simulink library "casper_library_pfbs"  (Simulink 7.2)
settings: Solver=ode45  SolverMode=SingleTasking  StartTime=0.0  StopTime=10.0  RelTol=1e-3
undefined symbols (not defined in the file or in its folder): pfb_coeff_gen_calc
libraries: xbsIndex_r4 x138, casper_library_pfbs x18, casper_library_delays x9, casper_library_misc x7, casper_library_flow_control x2
(part 2 of 3)

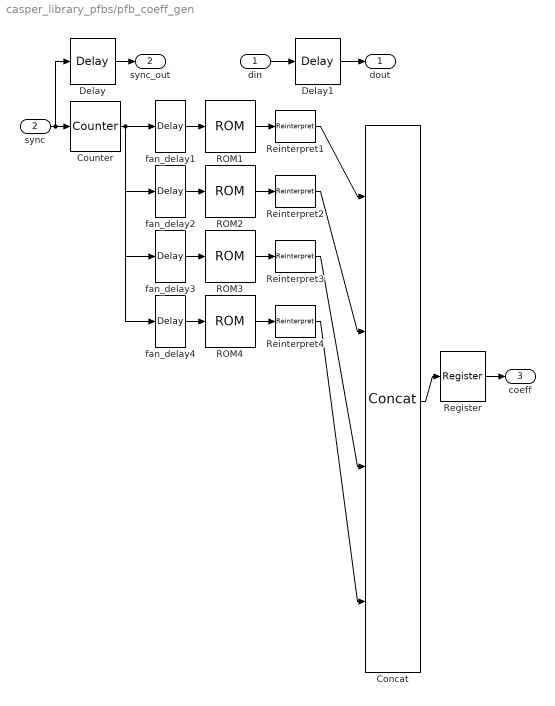
== system casper_library_pfbs/pfb_coeff_gen ==
  din : Inport
  sync : Inport  Port=2
  Concat : xbsIndex_r4/Concat  num_inputs=4  dbl_ovrd=off  block_type=concat
      settings: block_version=9.1.01
  Counter : xbsIndex_r4/Counter  cnt_type=Free Running  cnt_to=Inf  operation=Up  start_count=0  cnt_by_val=1  arith_type=Unsigned  n_bits=2  bin_pt=0  load_pin=off  rst=on  en=off  explicit_period=on  period=1  dbl_ovrd=off  use_behavioral_HDL=off  implementation=Fabric  use_rpm=on  block_type=counter
      settings: xl_area=[0, 0, 0, 0, 0, 0, 0]  block_version=9.1.01
  Delay : xbsIndex_r4/Delay  rst=off  infoeditControl=Selection of Reset will increase slice count due to use of real FFs and instead of SRLs  en=off  latency=bram_latency+1+fan_latency  dbl_ovrd=off  reg_retiming=off  block_type=delay
      settings: xl_area=[0, 0, 0, 0, 0, 0, 0]  block_version=9.1.01
  Delay1 : xbsIndex_r4/Delay  rst=off  infoeditControl=Selection of Reset will increase slice count due to use of real FFs and instead of SRLs  en=off  latency=bram_latency+1+fan_latency  dbl_ovrd=off  reg_retiming=off  block_type=delay
      settings: xl_area=[0, 0, 0, 0, 0, 0, 0]  block_version=9.1.01
  ROM1 : xbsIndex_r4/ROM  depth=4  initVector=pfb_coeff_gen_calc(2, 4,'hamming',0, 0,1,1,false)  distributed_mem=Block RAM  rst=off  init_reg=0  en=off  latency=bram_latency  gui_display_data_type=Fixed-point  arith_type="Signed  (2's comp)"  n_bits=8  bin_pt=7  preci_type=Single  exp_width=8  frac_width=24  dbl_ovrd=off  optimize=Area  use_rpm=on  block_type=sprom
      settings: xl_area=[0, 0, 0, 0, 0, 0, 0]
  ROM2 : xbsIndex_r4/ROM  depth=4  initVector=pfb_coeff_gen_calc(2, 4,'hamming',0, 0,1,2,false)  distributed_mem=Block RAM  rst=off  init_reg=0  en=off  latency=bram_latency  gui_display_data_type=Fixed-point  arith_type="Signed  (2's comp)"  n_bits=8  bin_pt=7  preci_type=Single  exp_width=8  frac_width=24  dbl_ovrd=off  optimize=Area  use_rpm=on  block_type=sprom
      settings: xl_area=[0, 0, 0, 0, 0, 0, 0]
  ROM3 : xbsIndex_r4/ROM  depth=4  initVector=pfb_coeff_gen_calc(2, 4,'hamming',0, 0,1,3,false)  distributed_mem=Block RAM  rst=off  init_reg=0  en=off  latency=bram_latency  gui_display_data_type=Fixed-point  arith_type="Signed  (2's comp)"  n_bits=8  bin_pt=7  preci_type=Single  exp_width=8  frac_width=24  dbl_ovrd=off  optimize=Area  use_rpm=on  block_type=sprom
      settings: xl_area=[0, 0, 0, 0, 0, 0, 0]
  ROM4 : xbsIndex_r4/ROM  depth=4  initVector=pfb_coeff_gen_calc(2, 4,'hamming',0, 0,1,4,false)  distributed_mem=Block RAM  rst=off  init_reg=0  en=off  latency=bram_latency  gui_display_data_type=Fixed-point  arith_type="Signed  (2's comp)"  n_bits=8  bin_pt=7  preci_type=Single  exp_width=8  frac_width=24  dbl_ovrd=off  optimize=Area  use_rpm=on  block_type=sprom
      settings: xl_area=[0, 0, 0, 0, 0, 0, 0]
  Register : xbsIndex_r4/Register  init=0  rst=off  en=off  dbl_ovrd=off  block_type=register
      settings: xl_area=[0, 0, 0, 0, 0, 0, 0]  block_version=9.1.01
  Reinterpret{1..4} (4 alike) : xbsIndex_r4/Reinterpret  force_arith_type=on  arith_type=Unsigned  force_bin_pt=on  bin_pt=0  block_type=reinterpret
      settings: infoedit="Changes signal type without altering the binary representation.   You can changed the signal between signed and unsigned, and relocate the binary point.<P><P>Hardware notes: In hardware this block costs nothing.<P><P>Example:  Suppose the input is 6 bits wide, signed, with 2 fractional bits, and the output is forced to unsigned with 0 fractional bits.  Then an input of -2.0 (1110.00 in binary 2's complement) becomes an output of 56 (111000 in binary)."  block_version=9.1.01
  fan_delay{1..4} (4 alike) : xbsIndex_r4/Delay  rst=off  infoeditControl=Selection of Reset will increase slice count due to use of real FFs and instead of SRLs  en=off  latency=fan_latency  dbl_ovrd=off  reg_retiming=off  block_type=delay
      settings: block_version=11.4
  dout : Outport
  sync_out : Outport  Port=2
  coeff : Outport  Port=3
  wires:
  din/1 -> Delay1/1
  Delay1/1 -> dout/1
  sync/1 -> Counter/1, Delay/1
  Delay/1 -> sync_out/1
  Concat/1 -> Register/1
  Register/1 -> coeff/1
  Counter/1 -> fan_delay1/1, fan_delay2/1, fan_delay3/1, fan_delay4/1
  fan_delay1/1 -> ROM1/1
  ROM1/1 -> Reinterpret1/1
  Reinterpret1/1 -> Concat/1
  fan_delay2/1 -> ROM2/1
  ROM2/1 -> Reinterpret2/1
  Reinterpret2/1 -> Concat/2
  fan_delay3/1 -> ROM3/1
  ROM3/1 -> Reinterpret3/1
  Reinterpret3/1 -> Concat/3
  fan_delay4/1 -> ROM4/1
  ROM4/1 -> Reinterpret4/1
  Reinterpret4/1 -> Concat/4

== system casper_library_pfbs/pfb_fir ==
  sync : Inport
  pol1_in1 : Inport  Port=2
  pol1_in2 : Inport  Port=3
  pol1_in1_coeffs : casper_library_pfbs/pfb_coeff_gen  PFBSize=5  CoeffBitWidth=18  TotalTaps=2  CoeffDistMem=off  WindowType=hamming  bram_latency=2  n_inputs=1  nput=0  fwidth=1  debug_mode=off  fan_latency=1
      settings: AttributesFormatString=|
      | PFBSize=5, n_inputs=1,
      | taps=2, input=0
  pol1_in1_first_tap : casper_library_pfbs/first_tap  PFBSize=5  CoeffBitWidth=18  TotalTaps=2  BitWidthIn=8  WindowType=hamming  mult_latency=2  bram_latency=2  n_inputs=1  fwidth=1  use_hdl=on  use_embedded=off
      settings: AttributesFormatString=taps=2
  pol1_in1_last_tap : casper_library_pfbs/last_tap  TotalTaps=2  BitWidthIn=8  BitWidthOut=18  CoeffBitWidth=18  add_latency=1  mult_latency=2  quantization="Round  (unbiased: Even Values)"  use_hdl=on  use_embedded=off
      link override pfb_add_tree/adder_tree1/addr1: latency=1  precision=User Defined  arith_type="Signed  (2's comp)"  n_bits=26  bin_pt=24  quantization=Truncate  overflow=Wrap  use_behavioral_HDL=off  hw_selection=Fabric  pipelined=on  use_rpm=on
      link override pfb_add_tree/adder_tree1/addr3: latency=1  precision=User Defined  arith_type="Signed  (2's comp)"  n_bits=26  bin_pt=24  quantization=Truncate  overflow=Wrap  use_behavioral_HDL=off  hw_selection=Fabric  pipelined=on  use_rpm=on
      link override pfb_add_tree/adder_tree2/addr1: latency=1  precision=User Defined  arith_type="Signed  (2's comp)"  n_bits=26  bin_pt=24  quantization=Truncate  overflow=Wrap  use_behavioral_HDL=off  hw_selection=Fabric  pipelined=on  use_rpm=on
      link override pfb_add_tree/adder_tree2/addr3: latency=1  precision=User Defined  arith_type="Signed  (2's comp)"  n_bits=26  bin_pt=24  quantization=Truncate  overflow=Wrap  use_behavioral_HDL=off  hw_selection=Fabric  pipelined=on  use_rpm=on
      link override pfb_add_tree/convert1: arith_type="Signed  (2's comp)"  n_bits=18  bin_pt=17  quantization="Round  (unbiased: Even Values)"  overflow=Wrap  latency=1  pipeline=on
      link override pfb_add_tree/convert2: arith_type="Signed  (2's comp)"  n_bits=18  bin_pt=17  quantization="Round  (unbiased: Even Values)"  overflow=Wrap  latency=1
      link override pfb_add_tree/scale1: scale_factor=-1
      link override pfb_add_tree/scale2: scale_factor=-1
      settings: AttributesFormatString=taps=2
  pol1_in2_coeffs : casper_library_pfbs/pfb_coeff_gen  PFBSize=5  CoeffBitWidth=18  TotalTaps=2  CoeffDistMem=off  WindowType=hamming  bram_latency=2  n_inputs=1  nput=1  fwidth=1  debug_mode=off  fan_latency=1
      settings: AttributesFormatString=|
      | PFBSize=5, n_inputs=1,
      | taps=2, input=1
  pol1_in2_first_tap : casper_library_pfbs/first_tap  PFBSize=5  CoeffBitWidth=18  TotalTaps=2  BitWidthIn=8  WindowType=hamming  mult_latency=2  bram_latency=2  n_inputs=1  fwidth=1  use_hdl=on  use_embedded=off
      settings: AttributesFormatString=taps=2
  pol1_in2_last_tap : casper_library_pfbs/last_tap  TotalTaps=2  BitWidthIn=8  BitWidthOut=18  CoeffBitWidth=18  add_latency=1  mult_latency=2  quantization="Round  (unbiased: Even Values)"  use_hdl=on  use_embedded=off
      link override pfb_add_tree/adder_tree1/addr1: latency=1  precision=User Defined  arith_type="Signed  (2's comp)"  n_bits=26  bin_pt=24  quantization=Truncate  overflow=Wrap  use_behavioral_HDL=off  hw_selection=Fabric  pipelined=on  use_rpm=on
      link override pfb_add_tree/adder_tree1/addr3: latency=1  precision=User Defined  arith_type="Signed  (2's comp)"  n_bits=26  bin_pt=24  quantization=Truncate  overflow=Wrap  use_behavioral_HDL=off  hw_selection=Fabric  pipelined=on  use_rpm=on
      link override pfb_add_tree/adder_tree2/addr1: latency=1  precision=User Defined  arith_type="Signed  (2's comp)"  n_bits=26  bin_pt=24  quantization=Truncate  overflow=Wrap  use_behavioral_HDL=off  hw_selection=Fabric  pipelined=on  use_rpm=on
      link override pfb_add_tree/adder_tree2/addr3: latency=1  precision=User Defined  arith_type="Signed  (2's comp)"  n_bits=26  bin_pt=24  quantization=Truncate  overflow=Wrap  use_behavioral_HDL=off  hw_selection=Fabric  pipelined=on  use_rpm=on
      link override pfb_add_tree/convert1: arith_type="Signed  (2's comp)"  n_bits=18  bin_pt=17  quantization="Round  (unbiased: Even Values)"  overflow=Wrap  latency=1  pipeline=on
      link override pfb_add_tree/convert2: arith_type="Signed  (2's comp)"  n_bits=18  bin_pt=17  quantization="Round  (unbiased: Even Values)"  overflow=Wrap  latency=1
      link override pfb_add_tree/scale1: scale_factor=-1
      link override pfb_add_tree/scale2: scale_factor=-1
      settings: AttributesFormatString=taps=2
  sync_out : Outport
  pol1_out1 : Outport  Port=2
  pol1_out2 : Outport  Port=3
  wires:
  pol1_in1/1 -> pol1_in1_coeffs/1
  sync/1 -> pol1_in1_coeffs/2, pol1_in2_coeffs/2
  pol1_in1_coeffs/1 -> pol1_in1_first_tap/1
  pol1_in1_coeffs/2 -> pol1_in1_first_tap/2, pol1_in2_first_tap/2
  pol1_in1_coeffs/3 -> pol1_in1_first_tap/3
  pol1_in1_first_tap/1 -> pol1_in1_last_tap/1
  pol1_in1_first_tap/2 -> pol1_in1_last_tap/2
  pol1_in1_first_tap/3 -> pol1_in1_last_tap/3
  pol1_in1_first_tap/4 -> pol1_in1_last_tap/4
  pol1_in1_last_tap/1 -> pol1_out1/1
  pol1_in1_last_tap/2 -> sync_out/1
  pol1_in2/1 -> pol1_in2_coeffs/1
  pol1_in2_coeffs/1 -> pol1_in2_first_tap/1
  pol1_in2_coeffs/3 -> pol1_in2_first_tap/3
  pol1_in2_first_tap/1 -> pol1_in2_last_tap/1
  pol1_in2_first_tap/2 -> pol1_in2_last_tap/2
  pol1_in2_first_tap/3 -> pol1_in2_last_tap/3
  pol1_in2_first_tap/4 -> pol1_in2_last_tap/4
  pol1_in2_last_tap/1 -> pol1_out2/1

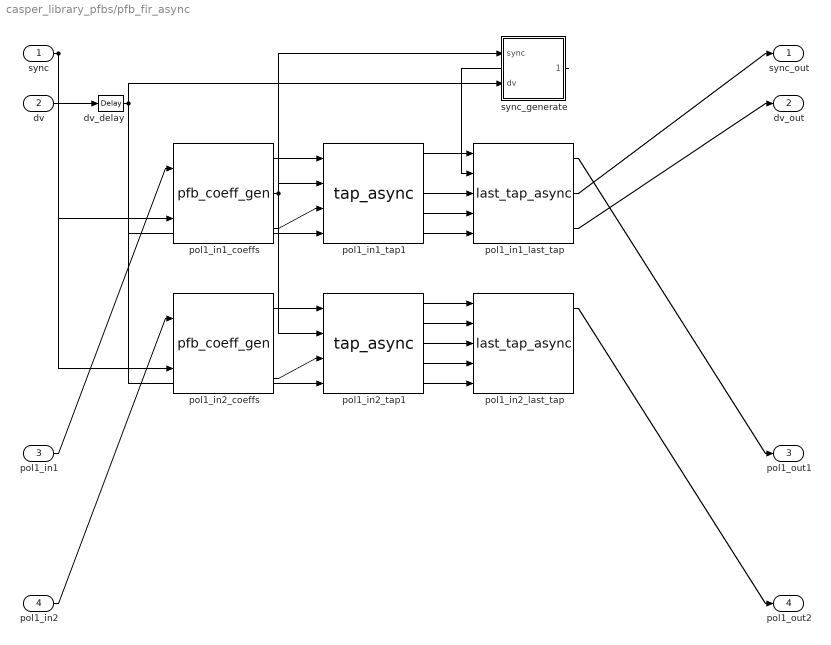
== system casper_library_pfbs/pfb_fir_async ==
  sync : Inport
  dv : Inport  Port=2
  pol1_in1 : Inport  Port=3
  pol1_in2 : Inport  Port=4
  dv_delay : xbsIndex_r4/Delay  rst=off  infoeditControl=Selection of Reset will increase slice count due to use of real FFs and instead of SRLs  en=off  latency=bram_latency+1  dbl_ovrd=off  reg_retiming=off  block_type=delay
      settings: block_version=11.4
  pol1_in1_coeffs : casper_library_pfbs/pfb_coeff_gen  PFBSize=5  CoeffBitWidth=8  TotalTaps=2  CoeffDistMem=off  WindowType=hamming  bram_latency=3  n_inputs=1  nput=0  fwidth=1  debug_mode=off  fan_latency=1
      settings: AttributesFormatString=|
      | PFBSize=5, n_inputs=1,
      | taps=2, input=0
  pol1_in1_last_tap : casper_library_pfbs/last_tap_async  input_num=1  total_taps=2  data_in_bits=8  data_out_bits=18  coeff_bits=8  add_latency=1  mult_latency=2  quantization=Truncate  use_hdl=on  use_embedded=off  async=on  debug_mode=off
      link override pfb_add_tree_async/adder_tree1/addr1: latency=1  precision=User Defined  arith_type="Signed  (2's comp)"  n_bits=16  bin_pt=14  quantization=Truncate  overflow=Wrap  use_behavioral_HDL=off  hw_selection=Fabric  pipelined=on  use_rpm=on
      link override pfb_add_tree_async/adder_tree1/addr3: latency=1  precision=User Defined  arith_type="Signed  (2's comp)"  n_bits=16  bin_pt=14  quantization=Truncate  overflow=Wrap  use_behavioral_HDL=off  hw_selection=Fabric  pipelined=on  use_rpm=on
      link override pfb_add_tree_async/adder_tree2/addr1: latency=1  precision=User Defined  arith_type="Signed  (2's comp)"  n_bits=16  bin_pt=14  quantization=Truncate  overflow=Wrap  use_behavioral_HDL=off  hw_selection=Fabric  pipelined=on  use_rpm=on
      link override pfb_add_tree_async/adder_tree2/addr3: latency=1  precision=User Defined  arith_type="Signed  (2's comp)"  n_bits=16  bin_pt=14  quantization=Truncate  overflow=Wrap  use_behavioral_HDL=off  hw_selection=Fabric  pipelined=on  use_rpm=on
      link override pfb_add_tree_async/convert1: arith_type="Signed  (2's comp)"  n_bits=data_out_bits  bin_pt=data_out_bits-1  quantization=Truncate  overflow=Wrap  latency=add_latency  pipeline=on
      link override pfb_add_tree_async/convert2: arith_type="Signed  (2's comp)"  n_bits=data_out_bits  bin_pt=data_out_bits-1  quantization=Truncate  overflow=Wrap  latency=add_latency  pipeline=on
      link override pfb_add_tree_async/scale1: scale_factor=-1
      link override pfb_add_tree_async/scale2: scale_factor=-1
      settings: AttributesFormatString=input(1), tap(2,2)
  pol1_in1_tap1 : casper_library_pfbs/tap_async  this_tap=1  pfb_bits=5  coeff_bits=8  total_taps=2  data_in_bits=8  mult_latency=2  bram_latency=3  simul_bits=1  fwidth=1  use_hdl=on  use_embedded=off  async=on  debug_mode=off
      settings: AttributesFormatString=tap(1/2)
  pol1_in2_coeffs : casper_library_pfbs/pfb_coeff_gen  PFBSize=5  CoeffBitWidth=8  TotalTaps=2  CoeffDistMem=off  WindowType=hamming  bram_latency=3  n_inputs=1  nput=1  fwidth=1  debug_mode=off  fan_latency=1
      settings: AttributesFormatString=|
      | PFBSize=5, n_inputs=1,
      | taps=2, input=1
  pol1_in2_last_tap : casper_library_pfbs/last_tap_async  input_num=2  total_taps=2  data_in_bits=8  data_out_bits=18  coeff_bits=8  add_latency=1  mult_latency=2  quantization=Truncate  use_hdl=on  use_embedded=off  async=on  debug_mode=off
      link override pfb_add_tree_async/adder_tree1/addr1: latency=1  precision=User Defined  arith_type="Signed  (2's comp)"  n_bits=16  bin_pt=14  quantization=Truncate  overflow=Wrap  use_behavioral_HDL=off  hw_selection=Fabric  pipelined=on  use_rpm=on
      link override pfb_add_tree_async/adder_tree1/addr3: latency=1  precision=User Defined  arith_type="Signed  (2's comp)"  n_bits=16  bin_pt=14  quantization=Truncate  overflow=Wrap  use_behavioral_HDL=off  hw_selection=Fabric  pipelined=on  use_rpm=on
      link override pfb_add_tree_async/adder_tree2/addr1: latency=1  precision=User Defined  arith_type="Signed  (2's comp)"  n_bits=16  bin_pt=14  quantization=Truncate  overflow=Wrap  use_behavioral_HDL=off  hw_selection=Fabric  pipelined=on  use_rpm=on
      link override pfb_add_tree_async/adder_tree2/addr3: latency=1  precision=User Defined  arith_type="Signed  (2's comp)"  n_bits=16  bin_pt=14  quantization=Truncate  overflow=Wrap  use_behavioral_HDL=off  hw_selection=Fabric  pipelined=on  use_rpm=on
      link override pfb_add_tree_async/convert1: arith_type="Signed  (2's comp)"  n_bits=data_out_bits  bin_pt=data_out_bits-1  quantization=Truncate  overflow=Wrap  latency=add_latency  pipeline=on
      link override pfb_add_tree_async/convert2: arith_type="Signed  (2's comp)"  n_bits=data_out_bits  bin_pt=data_out_bits-1  quantization=Truncate  overflow=Wrap  latency=add_latency  pipeline=on
      link override pfb_add_tree_async/scale1: scale_factor=-1
      link override pfb_add_tree_async/scale2: scale_factor=-1
      settings: AttributesFormatString=input(2), tap(2,2)
  pol1_in2_tap1 : casper_library_pfbs/tap_async  this_tap=1  pfb_bits=5  coeff_bits=8  total_taps=2  data_in_bits=8  mult_latency=2  bram_latency=3  simul_bits=1  fwidth=1  use_hdl=on  use_embedded=off  async=on  debug_mode=off
      settings: AttributesFormatString=tap(1/2)
  sync_generate : Subsystem
  sync_out : Outport
  dv_out : Outport  Port=2
  pol1_out1 : Outport  Port=3
  pol1_out2 : Outport  Port=4
  wires:
  dv/1 -> dv_delay/1
  pol1_in1/1 -> pol1_in1_coeffs/1
  sync/1 -> pol1_in1_coeffs/2, pol1_in2_coeffs/2
  pol1_in2/1 -> pol1_in2_coeffs/1
  pol1_in1_coeffs/1 -> pol1_in1_tap1/1
  pol1_in1_coeffs/2 -> pol1_in1_tap1/2, pol1_in2_tap1/2, sync_generate/1(sync)
  pol1_in1_coeffs/3 -> pol1_in1_tap1/3
  dv_delay/1 -> pol1_in1_tap1/4, pol1_in2_tap1/4, sync_generate/2(dv)
  pol1_in1_last_tap/1 -> pol1_out1/1
  pol1_in1_last_tap/2 -> sync_out/1
  pol1_in1_last_tap/3 -> dv_out/1
  pol1_in1_tap1/1 -> pol1_in1_last_tap/1
  pol1_in1_tap1/3 -> pol1_in1_last_tap/3
  pol1_in1_tap1/4 -> pol1_in1_last_tap/4
  pol1_in1_tap1/5 -> pol1_in1_last_tap/5
  pol1_in2_coeffs/1 -> pol1_in2_tap1/1
  pol1_in2_coeffs/3 -> pol1_in2_tap1/3
  pol1_in2_last_tap/1 -> pol1_out2/1
  pol1_in2_tap1/1 -> pol1_in2_last_tap/1
  pol1_in2_tap1/2 -> pol1_in2_last_tap/2
  pol1_in2_tap1/3 -> pol1_in2_last_tap/3
  pol1_in2_tap1/4 -> pol1_in2_last_tap/4
  pol1_in2_tap1/5 -> pol1_in2_last_tap/5
  sync_generate/1(sync_out) -> pol1_in1_last_tap/2

== system casper_library_pfbs/pfb_fir_coeff_gen ==

== system casper_library_pfbs/pfb_fir_generic ==

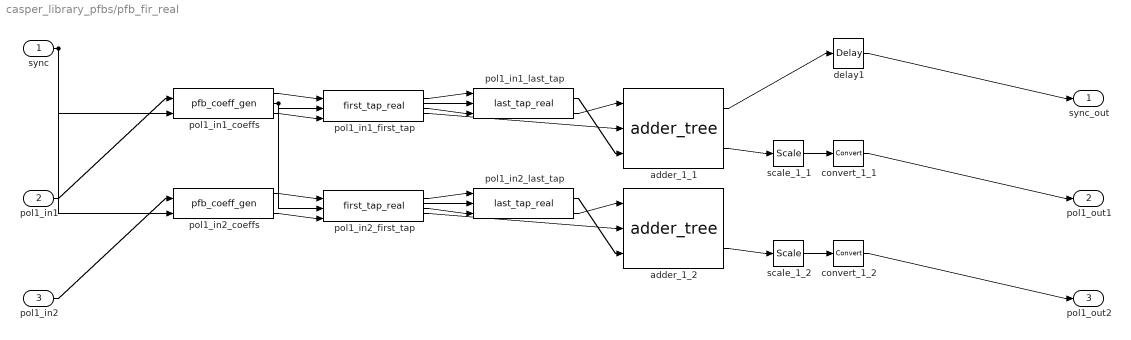
== system casper_library_pfbs/pfb_fir_real ==
  sync : Inport
  pol1_in1 : Inport  Port=2
  pol1_in2 : Inport  Port=3
  adder_1_1 : casper_library_misc/adder_tree  n_inputs=2  latency=1  adder_imp=Fabric  first_stage_hdl=on
      link override addr1: latency=1  precision=User Defined  arith_type="Signed  (2's comp)"  n_bits=26  bin_pt=24  quantization=Truncate  overflow=Wrap  use_behavioral_HDL=on  hw_selection=Fabric  pipelined=on  use_rpm=on
      link override addr3: latency=1  precision=User Defined  arith_type="Signed  (2's comp)"  n_bits=26  bin_pt=24  quantization=Truncate  overflow=Wrap  use_behavioral_HDL=off  hw_selection=Fabric  pipelined=on  use_rpm=on
      settings: AttributesFormatString=latency 1
  adder_1_2 : casper_library_misc/adder_tree  n_inputs=2  latency=1  adder_imp=Fabric  first_stage_hdl=on
      link override addr1: latency=1  precision=User Defined  arith_type="Signed  (2's comp)"  n_bits=26  bin_pt=24  quantization=Truncate  overflow=Wrap  use_behavioral_HDL=on  hw_selection=Fabric  pipelined=on  use_rpm=on
      link override addr3: latency=1  precision=User Defined  arith_type="Signed  (2's comp)"  n_bits=26  bin_pt=24  quantization=Truncate  overflow=Wrap  use_behavioral_HDL=off  hw_selection=Fabric  pipelined=on  use_rpm=on
      settings: AttributesFormatString=latency 1
  convert_1_1 : xbsIndex_r4/Convert  gui_display_data_type=Fixed-point  arith_type="Signed  (2's comp)"  n_bits=18  bin_pt=17  float_type=Single  exp_bits=8  fraction_bits=24  quantization="Round  (unbiased: Even Values)"  overflow=Wrap  en=off  latency=1  dbl_ovrd=off  pipeline=on  block_type=convert
  convert_1_2 : xbsIndex_r4/Convert  gui_display_data_type=Fixed-point  arith_type="Signed  (2's comp)"  n_bits=18  bin_pt=17  float_type=Single  exp_bits=8  fraction_bits=24  quantization="Round  (unbiased: Even Values)"  overflow=Wrap  en=off  latency=1  dbl_ovrd=off  pipeline=on  block_type=convert
  delay1 : xbsIndex_r4/Delay  rst=off  infoeditControl=Selection of Reset will increase slice count due to use of real FFs and instead of SRLs  en=off  latency=1  dbl_ovrd=off  reg_retiming=off  block_type=delay
  pol1_in1_coeffs : casper_library_pfbs/pfb_coeff_gen  PFBSize=5  CoeffBitWidth=18  TotalTaps=2  CoeffDistMem=off  WindowType=hamming  bram_latency=2  n_inputs=1  nput=0  fwidth=1  debug_mode=off  fan_latency=1
      settings: AttributesFormatString=|
      | PFBSize=5, n_inputs=1,
      | taps=2, input=0
  pol1_in1_first_tap : casper_library_pfbs/first_tap_real  PFBSize=5  CoeffBitWidth=18  TotalTaps=2  BitWidthIn=8  WindowType=hamming  mult_latency=2  bram_latency=2  n_inputs=1  fwidth=1  use_hdl=on  use_embedded=off
      settings: AttributesFormatString=taps=2
  pol1_in1_last_tap : casper_library_pfbs/last_tap_real  BitWidthIn=8  CoeffBitWidth=18  mult_latency=2  use_hdl=on  use_embedded=off
  pol1_in2_coeffs : casper_library_pfbs/pfb_coeff_gen  PFBSize=5  CoeffBitWidth=18  TotalTaps=2  CoeffDistMem=off  WindowType=hamming  bram_latency=2  n_inputs=1  nput=1  fwidth=1  debug_mode=off  fan_latency=1
      settings: AttributesFormatString=|
      | PFBSize=5, n_inputs=1,
      | taps=2, input=1
  pol1_in2_first_tap : casper_library_pfbs/first_tap_real  PFBSize=5  CoeffBitWidth=18  TotalTaps=2  BitWidthIn=8  WindowType=hamming  mult_latency=2  bram_latency=2  n_inputs=1  fwidth=1  use_hdl=on  use_embedded=off
      settings: AttributesFormatString=taps=2
  pol1_in2_last_tap : casper_library_pfbs/last_tap_real  BitWidthIn=8  CoeffBitWidth=18  mult_latency=2  use_hdl=on  use_embedded=off
  scale_1_1 : xbsIndex_r4/Scale  scale_factor=-1  dbl_ovrd=off  block_type=scale
  scale_1_2 : xbsIndex_r4/Scale  scale_factor=-1  dbl_ovrd=off  block_type=scale
  sync_out : Outport
  pol1_out1 : Outport  Port=2
  pol1_out2 : Outport  Port=3
  wires:
  pol1_in1/1 -> pol1_in1_coeffs/1
  sync/1 -> pol1_in1_coeffs/2, pol1_in2_coeffs/2
  pol1_in1_coeffs/1 -> pol1_in1_first_tap/1
  pol1_in1_coeffs/2 -> pol1_in1_first_tap/2, pol1_in2_first_tap/2
  pol1_in1_coeffs/3 -> pol1_in1_first_tap/3
  pol1_in2/1 -> pol1_in2_coeffs/1
  pol1_in2_coeffs/1 -> pol1_in2_first_tap/1
  pol1_in2_coeffs/3 -> pol1_in2_first_tap/3
  adder_1_1/1 -> delay1/1
  delay1/1 -> sync_out/1
  adder_1_1/2 -> scale_1_1/1
  scale_1_1/1 -> convert_1_1/1
  convert_1_1/1 -> pol1_out1/1
  adder_1_2/2 -> scale_1_2/1
  scale_1_2/1 -> convert_1_2/1
  convert_1_2/1 -> pol1_out2/1
  pol1_in1_last_tap/2 -> adder_1_1/1
  pol1_in1_last_tap/1 -> adder_1_1/3
  pol1_in1_first_tap/1 -> pol1_in1_last_tap/1
  pol1_in1_first_tap/2 -> pol1_in1_last_tap/2
  pol1_in1_first_tap/3 -> pol1_in1_last_tap/3
  pol1_in1_first_tap/4 -> adder_1_1/2
  pol1_in2_last_tap/2 -> adder_1_2/1
  pol1_in2_last_tap/1 -> adder_1_2/3
  pol1_in2_first_tap/1 -> pol1_in2_last_tap/1
  pol1_in2_first_tap/2 -> pol1_in2_last_tap/2
  pol1_in2_first_tap/3 -> pol1_in2_last_tap/3
  pol1_in2_first_tap/4 -> adder_1_2/2

== system casper_library_pfbs/pfb_fir_taps ==

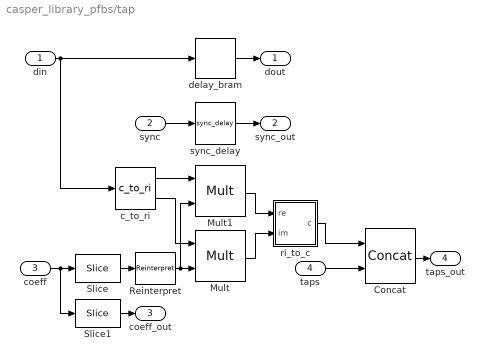
== system casper_library_pfbs/tap ==
  din : Inport
  sync : Inport  Port=2
  coeff : Inport  Port=3
  taps : Inport  Port=4
  Concat : xbsIndex_r4/Concat  num_inputs=2  dbl_ovrd=off  block_type=concat
      settings: block_version=9.1.01
  Mult : xbsIndex_r4/Mult  precision=Full  arith_type="Signed  (2's comp)"  n_bits=8  bin_pt=2  quantization=Truncate  overflow=Wrap  en=off  latency=mult_latency  dbl_ovrd=off  use_behavioral_HDL=off  opt=Speed  use_embedded=on  optimum_pipeline=off  pipeline=on  use_rpm=on  placement_style=Rectangular shape  block_type=mult
      settings: infoedit=Hardware notes: To use the internal pipeline stage of the dedicated multiplier you must select 'Pipeline for maximum performance'.  xl_area=[0, 0, 0, 0, 0, 0, 0]  block_version=9.1.01
  Mult1 : xbsIndex_r4/Mult  precision=Full  arith_type="Signed  (2's comp)"  n_bits=8  bin_pt=2  quantization=Truncate  overflow=Wrap  en=off  latency=mult_latency  dbl_ovrd=off  use_behavioral_HDL=off  opt=Speed  use_embedded=on  optimum_pipeline=off  pipeline=on  use_rpm=on  placement_style=Rectangular shape  block_type=mult
      settings: infoedit=Hardware notes: To use the internal pipeline stage of the dedicated multiplier you must select 'Pipeline for maximum performance'.  xl_area=[0, 0, 0, 0, 0, 0, 0]  block_version=9.1.01
  Reinterpret : xbsIndex_r4/Reinterpret  force_arith_type=on  arith_type="Signed  (2's comp)"  force_bin_pt=on  bin_pt=coeff_frac_width  block_type=reinterpret
      settings: infoedit="Changes signal type without altering the binary representation.   You can changed the signal between signed and unsigned, and relocate the binary point.<P><P>Hardware notes: In hardware this block costs nothing.<P><P>Example:  Suppose the input is 6 bits wide, signed, with 2 fractional bits, and the output is forced to unsigned with 0 fractional bits.  Then an input of -2.0 (1110.00 in binary 2's complement) becomes an output of 56 (111000 in binary)."  block_version=9.1.01
  Slice : xbsIndex_r4/Slice  nbits=coeff_width  boolean_output=off  mode=Lower Bit Location + Width  bit1=0  base1=MSB of Input  bit0=0  base0=LSB of Input  dbl_ovrd=off  block_type=slice
      settings: infoedit="Extracts a given range of bits from each input sample and presents it at the output.  The output type is ordinarily unsigned with binary point at zero, but can be Boolean when the slice is one bit wide.<P><P>Hardware notes: In hardware this block costs nothing."  block_version=9.1.01
  Slice1 : xbsIndex_r4/Slice  nbits=0  boolean_output=off  mode=Two Bit Locations  bit1=0  base1=MSB of Input  bit0=coeff_width  base0=LSB of Input  dbl_ovrd=off  block_type=slice
      settings: infoedit="Extracts a given range of bits from each input sample and presents it at the output.  The output type is ordinarily unsigned with binary point at zero, but can be Boolean when the slice is one bit wide.<P><P>Hardware notes: In hardware this block costs nothing."  block_version=9.1.01
  c_to_ri : casper_library_misc/c_to_ri  n_bits=data_width  bin_pt=data_width-1
      settings: AttributesFormatString=_ r/i
  delay_bram : casper_library_delays/delay_bram  DelayLen=delay  bram_latency=bram_latency  use_dsp48=off  async=off
  ri_to_c : Subsystem
  sync_delay : casper_library_delays/sync_delay  DelayLen=delay
  dout : Outport
  sync_out : Outport  Port=2
  coeff_out : Outport  Port=3
  taps_out : Outport  Port=4
  wires:
  Reinterpret/1 -> Mult/2, Mult1/2
  Slice/1 -> Reinterpret/1
  Slice1/1 -> coeff_out/1
  coeff/1 -> Slice1/1, Slice/1
  Concat/1 -> taps_out/1
  taps/1 -> Concat/2
  sync_delay/1 -> sync_out/1
  sync/1 -> sync_delay/1
  Mult1/1 -> ri_to_c/1(re)
  Mult/1 -> ri_to_c/2(im)
  ri_to_c/1(c) -> Concat/1
  c_to_ri/1 -> Mult1/1
  c_to_ri/2 -> Mult/1
  din/1 -> delay_bram/1, c_to_ri/1
  delay_bram/1 -> dout/1

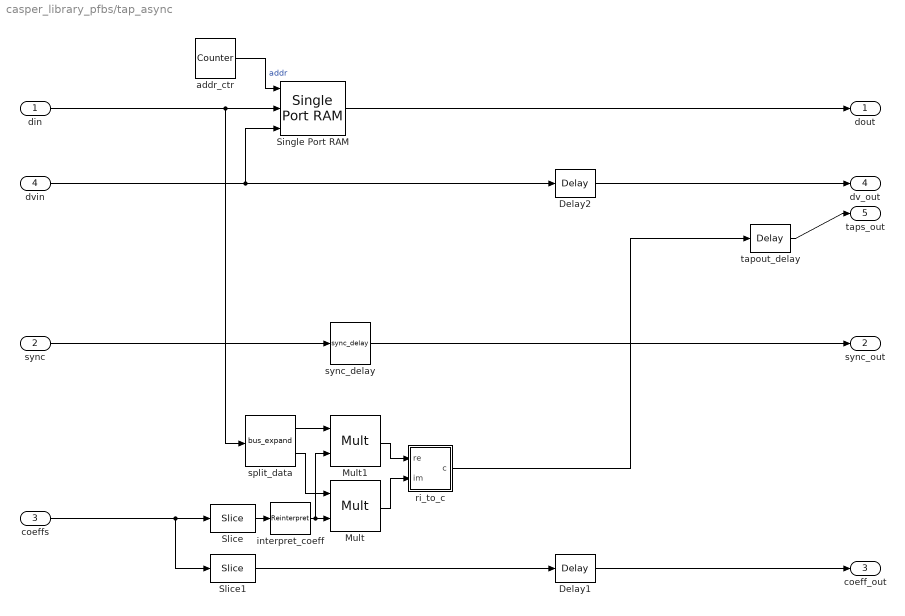
== system casper_library_pfbs/tap_async ==
  din : Inport
  sync : Inport  Port=2
  coeffs : Inport  Port=3
  dvin : Inport  Port=4
  Delay1 : xbsIndex_r4/Delay  rst=off  infoeditControl=Selection of Reset will increase slice count due to use of real FFs and instead of SRLs  en=off  latency=bram_latency  dbl_ovrd=off  reg_retiming=off  block_type=delay
      settings: block_version=11.4
  Delay2 : xbsIndex_r4/Delay  rst=off  infoeditControl=Selection of Reset will increase slice count due to use of real FFs and instead of SRLs  en=off  latency=bram_latency  dbl_ovrd=off  reg_retiming=off  block_type=delay
      settings: block_version=11.4
  Mult : xbsIndex_r4/Mult  precision=Full  arith_type="Signed  (2's comp)"  n_bits=8  bin_pt=2  quantization=Truncate  overflow=Wrap  en=off  latency=mult_latency  dbl_ovrd=off  use_behavioral_HDL=on  opt=Speed  use_embedded=off  optimum_pipeline=off  pipeline=on  use_rpm=on  placement_style=Rectangular shape  block_type=mult
      settings: infoedit=Hardware notes: To use the internal pipeline stage of the dedicated multiplier you must select 'Pipeline for maximum performance'.  xl_area=[0, 0, 0, 0, 0, 0, 0]  block_version=9.1.01
  Mult1 : xbsIndex_r4/Mult  precision=Full  arith_type="Signed  (2's comp)"  n_bits=8  bin_pt=2  quantization=Truncate  overflow=Wrap  en=off  latency=mult_latency  dbl_ovrd=off  use_behavioral_HDL=on  opt=Speed  use_embedded=off  optimum_pipeline=off  pipeline=on  use_rpm=on  placement_style=Rectangular shape  block_type=mult
      settings: infoedit=Hardware notes: To use the internal pipeline stage of the dedicated multiplier you must select 'Pipeline for maximum performance'.  xl_area=[0, 0, 0, 0, 0, 0, 0]  block_version=9.1.01
  Single Port RAM : xbsIndex_r4/Single Port RAM  depth=2^(pfb_bits - simul_bits)  initVector=0  distributed_mem=Block RAM  write_mode=Read Before Write  rst=off  init_reg=0  en=off  latency=bram_latency  dbl_ovrd=off  optimize=Area  block_type=spram
      settings: xl_area=[0, 0, 0, 0, 0, 0, 0]  block_version=9.1.01
  Slice : xbsIndex_r4/Slice  nbits=coeff_bits  boolean_output=off  mode=Lower Bit Location + Width  bit1=0  base1=MSB of Input  bit0=0  base0=LSB of Input  dbl_ovrd=off  block_type=slice
      settings: block_version=9.1.01
  Slice1 : xbsIndex_r4/Slice  nbits=coeff_bits * (total_taps - 1)  boolean_output=off  mode=Two Bit Locations  bit1=0  base1=MSB of Input  bit0=coeff_bits  base0=LSB of Input  dbl_ovrd=off  block_type=slice
      settings: block_version=9.1.01
  addr_ctr : xbsIndex_r4/Counter  cnt_type=Free Running  cnt_to=0  operation=Up  start_count=0  cnt_by_val=1  arith_type=Unsigned  n_bits=pfb_bits - simul_bits  bin_pt=0  load_pin=off  rst=off  en=off  explicit_period=on  period=1  dbl_ovrd=off  use_behavioral_HDL=off  implementation=Fabric  use_rpm=off  block_type=counter
      settings: xl_area=[0, 0, 0, 0, 0, 0, 0]  block_version=9.1.01
  interpret_coeff : xbsIndex_r4/Reinterpret  force_arith_type=on  arith_type="Signed  (2's comp)"  force_bin_pt=on  bin_pt=coeff_bits - 1  block_type=reinterpret
      settings: infoedit="Changes signal type without altering the binary representation.   You can changed the signal between signed and unsigned, and relocate the binary point.<br><br>Hardware notes: In hardware this block costs nothing.<br><br>Example:  Suppose the input is 6 bits wide, signed, with 2 fractional bits, and the output is forced to unsigned with 0 fractional bits.  Then an input of -2.0 (1110.00 in binary 2's complement) becomes an output of 56 (111000 in binary)."  block_version=9.1.01
  ri_to_c : Subsystem
  split_data : casper_library_flow_control/bus_expand  mode=divisions of equal size  outputNum=2  outputWidth=data_in_bits  outputBinaryPt=data_in_bits - 1  outputArithmeticType=1  show_format=off  outputToWorkspace=off  variablePrefix=out  outputToModelAsWell=on
      settings: AttributesFormatString=2 outputs
  sync_delay : casper_library_delays/sync_delay  DelayLen=2^(pfb_bits - simul_bits)
  tapout_delay : xbsIndex_r4/Delay  rst=off  infoeditControl=Selection of Reset will increase slice count due to use of real FFs and instead of SRLs  en=off  latency=bram_latency * (total_taps - this_tap)  dbl_ovrd=off  reg_retiming=off  block_type=delay
      settings: block_version=11.4
  dout : Outport
  sync_out : Outport  Port=2
  coeff_out : Outport  Port=3
  dv_out : Outport  Port=4
  taps_out : Outport  Port=5
  wires:
  coeffs/1 -> Slice1/1, Slice/1
  Mult/1 -> ri_to_c/2(im)
  Mult1/1 -> ri_to_c/1(re)
  split_data/2 -> Mult/1
  split_data/1 -> Mult1/1
  sync/1 -> sync_delay/1
  din/1 -> split_data/1, Single Port RAM/2
  sync_delay/1 -> sync_out/1
  Slice1/1 -> Delay1/1
  Slice/1 -> interpret_coeff/1
  interpret_coeff/1 -> Mult1/2, Mult/2
  addr_ctr/1 -> Single Port RAM/1  "addr"
  Single Port RAM/1 -> dout/1
  ri_to_c/1(c) -> tapout_delay/1
  dvin/1 -> Single Port RAM/3, Delay2/1
  Delay1/1 -> coeff_out/1
  Delay2/1 -> dv_out/1
  tapout_delay/1 -> taps_out/1

== system casper_library_pfbs/tap_real ==
  din : Inport
  sync : Inport  Port=2
  coeff : Inport  Port=3
  Mult : xbsIndex_r4/Mult  precision=Full  arith_type="Signed  (2's comp)"  n_bits=8  bin_pt=2  quantization=Truncate  overflow=Wrap  en=off  latency=mult_latency  dbl_ovrd=off  use_behavioral_HDL=on  opt=Speed  use_embedded=off  optimum_pipeline=off  pipeline=on  use_rpm=on  placement_style=Rectangular shape  block_type=mult
      settings: infoedit=Hardware notes: To use the internal pipeline stage of the dedicated multiplier you must select 'Pipeline for maximum performance'.  xl_area=[0, 0, 0, 0, 0, 0, 0]  block_version=9.1.01
  Reinterpret : xbsIndex_r4/Reinterpret  force_arith_type=on  arith_type="Signed  (2's comp)"  force_bin_pt=on  bin_pt=coeff_frac_width  block_type=reinterpret
      settings: infoedit="Changes signal type without altering the binary representation.   You can changed the signal between signed and unsigned, and relocate the binary point.<P><P>Hardware notes: In hardware this block costs nothing.<P><P>Example:  Suppose the input is 6 bits wide, signed, with 2 fractional bits, and the output is forced to unsigned with 0 fractional bits.  Then an input of -2.0 (1110.00 in binary 2's complement) becomes an output of 56 (111000 in binary)."  block_version=9.1.01
  Reinterpret1 : xbsIndex_r4/Reinterpret  force_arith_type=on  arith_type="Signed  (2's comp)"  force_bin_pt=on  bin_pt=data_width - 1  block_type=reinterpret
      settings: infoedit="Changes signal type without altering the binary representation.   You can changed the signal between signed and unsigned, and relocate the binary point.<P><P>Hardware notes: In hardware this block costs nothing.<P><P>Example:  Suppose the input is 6 bits wide, signed, with 2 fractional bits, and the output is forced to unsigned with 0 fractional bits.  Then an input of -2.0 (1110.00 in binary 2's complement) becomes an output of 56 (111000 in binary)."  block_version=9.1.01
  Slice : xbsIndex_r4/Slice  nbits=coeff_width  boolean_output=off  mode=Lower Bit Location + Width  bit1=0  base1=MSB of Input  bit0=0  base0=LSB of Input  dbl_ovrd=off  block_type=slice
      settings: infoedit="Extracts a given range of bits from each input sample and presents it at the output.  The output type is ordinarily unsigned with binary point at zero, but can be Boolean when the slice is one bit wide.<P><P>Hardware notes: In hardware this block costs nothing."  block_version=9.1.01
  Slice1 : xbsIndex_r4/Slice  nbits=0  boolean_output=off  mode=Two Bit Locations  bit1=0  base1=MSB of Input  bit0=coeff_width  base0=LSB of Input  dbl_ovrd=off  block_type=slice
      settings: infoedit="Extracts a given range of bits from each input sample and presents it at the output.  The output type is ordinarily unsigned with binary point at zero, but can be Boolean when the slice is one bit wide.<P><P>Hardware notes: In hardware this block costs nothing."  block_version=9.1.01
  delay_bram : casper_library_delays/delay_bram  DelayLen=delay  bram_latency=bram_latency  use_dsp48=off  async=off
  sync_delay : casper_library_delays/sync_delay  DelayLen=delay
  dout : Outport
  sync_out : Outport  Port=2
  coeff_out : Outport  Port=3
  taps_out : Outport  Port=4
  wires:
  Reinterpret1/1 -> Mult/1
  Reinterpret/1 -> Mult/2
  Slice/1 -> Reinterpret/1
  Slice1/1 -> coeff_out/1
  coeff/1 -> Slice1/1, Slice/1
  sync_delay/1 -> sync_out/1
  sync/1 -> sync_delay/1
  Mult/1 -> taps_out/1
  din/1 -> delay_bram/1, Reinterpret1/1
  delay_bram/1 -> dout/1

== system casper_library_pfbs/first_tap/ri_to_c ==
  re : Inport
  im : Inport  Port=2
  Concat : xbsIndex_r4/Concat  num_inputs=2  dbl_ovrd=off  block_type=concat
      settings: block_version=9.1.01
  Reinterpret : xbsIndex_r4/Reinterpret  force_arith_type=on  arith_type=Unsigned  force_bin_pt=on  bin_pt=0  block_type=reinterpret
      settings: infoedit="Changes signal type without altering the binary representation.   You can changed the signal between signed and unsigned, and relocate the binary point.<P><P>Hardware notes: In hardware this block costs nothing.<P><P>Example:  Suppose the input is 6 bits wide, signed, with 2 fractional bits, and the output is forced to unsigned with 0 fractional bits.  Then an input of -2.0 (1110.00 in binary 2's complement) becomes an output of 56 (111000 in binary)."  block_version=9.1.01
  Reinterpret1 : xbsIndex_r4/Reinterpret  force_arith_type=on  arith_type=Unsigned  force_bin_pt=on  bin_pt=0  block_type=reinterpret
      settings: infoedit="Changes signal type without altering the binary representation.   You can changed the signal between signed and unsigned, and relocate the binary point.<P><P>Hardware notes: In hardware this block costs nothing.<P><P>Example:  Suppose the input is 6 bits wide, signed, with 2 fractional bits, and the output is forced to unsigned with 0 fractional bits.  Then an input of -2.0 (1110.00 in binary 2's complement) becomes an output of 56 (111000 in binary)."  block_version=9.1.01
  c : Outport
  wires:
  im/1 -> Reinterpret1/1
  Concat/1 -> c/1
  re/1 -> Reinterpret/1
  Reinterpret1/1 -> Concat/2
  Reinterpret/1 -> Concat/1

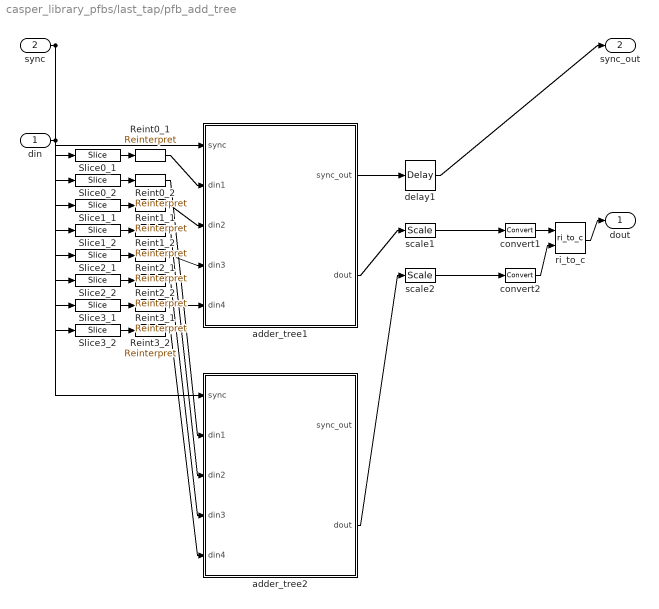
== system casper_library_pfbs/last_tap/pfb_add_tree ==
  din : Inport
  sync : Inport  Port=2
  Reint0_1 : xbsIndex_r4/Reinterpret  force_arith_type=on  arith_type="Signed  (2's comp)"  force_bin_pt=on  bin_pt=14  block_type=reinterpret
      settings: infoedit="Changes signal type without altering the binary representation.   You can changed the signal between signed and unsigned, and relocate the binary point.<br><br>Hardware notes: In hardware this block costs nothing.<br><br>Example:  Suppose the input is 6 bits wide, signed, with 2 fractional bits, and the output is forced to unsigned with 0 fractional bits.  Then an input of -2.0 (1110.00 in binary 2's complement) becomes an output of 56 (111000 in binary)."
  Reint0_2 : xbsIndex_r4/Reinterpret  force_arith_type=on  arith_type="Signed  (2's comp)"  force_bin_pt=on  bin_pt=14  block_type=reinterpret
      settings: infoedit="Changes signal type without altering the binary representation.   You can changed the signal between signed and unsigned, and relocate the binary point.<br><br>Hardware notes: In hardware this block costs nothing.<br><br>Example:  Suppose the input is 6 bits wide, signed, with 2 fractional bits, and the output is forced to unsigned with 0 fractional bits.  Then an input of -2.0 (1110.00 in binary 2's complement) becomes an output of 56 (111000 in binary)."
  Reint1_1 : xbsIndex_r4/Reinterpret  force_arith_type=on  arith_type="Signed  (2's comp)"  force_bin_pt=on  bin_pt=14  block_type=reinterpret
      settings: infoedit="Changes signal type without altering the binary representation.   You can changed the signal between signed and unsigned, and relocate the binary point.<br><br>Hardware notes: In hardware this block costs nothing.<br><br>Example:  Suppose the input is 6 bits wide, signed, with 2 fractional bits, and the output is forced to unsigned with 0 fractional bits.  Then an input of -2.0 (1110.00 in binary 2's complement) becomes an output of 56 (111000 in binary)."
  Reint1_2 : xbsIndex_r4/Reinterpret  force_arith_type=on  arith_type="Signed  (2's comp)"  force_bin_pt=on  bin_pt=14  block_type=reinterpret
      settings: infoedit="Changes signal type without altering the binary representation.   You can changed the signal between signed and unsigned, and relocate the binary point.<br><br>Hardware notes: In hardware this block costs nothing.<br><br>Example:  Suppose the input is 6 bits wide, signed, with 2 fractional bits, and the output is forced to unsigned with 0 fractional bits.  Then an input of -2.0 (1110.00 in binary 2's complement) becomes an output of 56 (111000 in binary)."
  Reint2_1 : xbsIndex_r4/Reinterpret  force_arith_type=on  arith_type="Signed  (2's comp)"  force_bin_pt=on  bin_pt=14  block_type=reinterpret
      settings: infoedit="Changes signal type without altering the binary representation.   You can changed the signal between signed and unsigned, and relocate the binary point.<br><br>Hardware notes: In hardware this block costs nothing.<br><br>Example:  Suppose the input is 6 bits wide, signed, with 2 fractional bits, and the output is forced to unsigned with 0 fractional bits.  Then an input of -2.0 (1110.00 in binary 2's complement) becomes an output of 56 (111000 in binary)."
  Reint2_2 : xbsIndex_r4/Reinterpret  force_arith_type=on  arith_type="Signed  (2's comp)"  force_bin_pt=on  bin_pt=14  block_type=reinterpret
      settings: infoedit="Changes signal type without altering the binary representation.   You can changed the signal between signed and unsigned, and relocate the binary point.<br><br>Hardware notes: In hardware this block costs nothing.<br><br>Example:  Suppose the input is 6 bits wide, signed, with 2 fractional bits, and the output is forced to unsigned with 0 fractional bits.  Then an input of -2.0 (1110.00 in binary 2's complement) becomes an output of 56 (111000 in binary)."
  Reint3_1 : xbsIndex_r4/Reinterpret  force_arith_type=on  arith_type="Signed  (2's comp)"  force_bin_pt=on  bin_pt=14  block_type=reinterpret
      settings: infoedit="Changes signal type without altering the binary representation.   You can changed the signal between signed and unsigned, and relocate the binary point.<br><br>Hardware notes: In hardware this block costs nothing.<br><br>Example:  Suppose the input is 6 bits wide, signed, with 2 fractional bits, and the output is forced to unsigned with 0 fractional bits.  Then an input of -2.0 (1110.00 in binary 2's complement) becomes an output of 56 (111000 in binary)."
  Reint3_2 : xbsIndex_r4/Reinterpret  force_arith_type=on  arith_type="Signed  (2's comp)"  force_bin_pt=on  bin_pt=14  block_type=reinterpret
      settings: infoedit="Changes signal type without altering the binary representation.   You can changed the signal between signed and unsigned, and relocate the binary point.<br><br>Hardware notes: In hardware this block costs nothing.<br><br>Example:  Suppose the input is 6 bits wide, signed, with 2 fractional bits, and the output is forced to unsigned with 0 fractional bits.  Then an input of -2.0 (1110.00 in binary 2's complement) becomes an output of 56 (111000 in binary)."
  Slice0_1 : xbsIndex_r4/Slice  nbits=16  boolean_output=off  mode=Upper Bit Location + Width  bit1=0  base1=MSB of Input  bit0=0  base0=MSB of Input  dbl_ovrd=off  block_type=slice
  Slice0_2 : xbsIndex_r4/Slice  nbits=16  boolean_output=off  mode=Upper Bit Location + Width  bit1=-16  base1=MSB of Input  bit0=0  base0=MSB of Input  dbl_ovrd=off  block_type=slice
  Slice1_1 : xbsIndex_r4/Slice  nbits=16  boolean_output=off  mode=Upper Bit Location + Width  bit1=-32  base1=MSB of Input  bit0=0  base0=MSB of Input  dbl_ovrd=off  block_type=slice
  Slice1_2 : xbsIndex_r4/Slice  nbits=16  boolean_output=off  mode=Upper Bit Location + Width  bit1=-48  base1=MSB of Input  bit0=0  base0=MSB of Input  dbl_ovrd=off  block_type=slice
  Slice2_1 : xbsIndex_r4/Slice  nbits=16  boolean_output=off  mode=Upper Bit Location + Width  bit1=-64  base1=MSB of Input  bit0=0  base0=MSB of Input  dbl_ovrd=off  block_type=slice
  Slice2_2 : xbsIndex_r4/Slice  nbits=16  boolean_output=off  mode=Upper Bit Location + Width  bit1=-80  base1=MSB of Input  bit0=0  base0=MSB of Input  dbl_ovrd=off  block_type=slice
  Slice3_1 : xbsIndex_r4/Slice  nbits=16  boolean_output=off  mode=Upper Bit Location + Width  bit1=-96  base1=MSB of Input  bit0=0  base0=MSB of Input  dbl_ovrd=off  block_type=slice
  Slice3_2 : xbsIndex_r4/Slice  nbits=16  boolean_output=off  mode=Upper Bit Location + Width  bit1=-112  base1=MSB of Input  bit0=0  base0=MSB of Input  dbl_ovrd=off  block_type=slice
  adder_tree1 : Subsystem  AncestorBlock=casper_library_misc/adder_tree  mask(adder_tree){n_inputs=4, latency=1, adder_imp=Fabric, first_stage_hdl=off}
      mask prompts: n_inputs "Number of Inputs"; latency "Add Latency"; adder_imp "Adder implementation"; first_stage_hdl "Use behavioural HDL for first stage of adders"
      mask help:
      | Sums all inputs using a tree of adds and delays.
      |
      | Number of inputs: The number of inputs to the block to be summed
      | Add latency: The number of clock cycles to perform one addition (affects timing)..
      | Adder implementation: choice of fabric or DSP48E core, or behavioral HDL
      | Use behavioural HDL for first stage of adders: Causes the first stage of adders to be absorbed into DSP blocks if multipliers precede them (Virtex 5). Overrides Adder implementation
      mask init:
      | adder_tree_init(gcb, ...
      |     'n_inputs', n_inputs, ...
      |     'latency', latency, ...
      |     'adder_imp', adder_imp, ...
      |     'first_stage_hdl', first_stage_hdl);
      settings: AttributesFormatString=latency 2
      mask Help: eval('xlWeb(''http://casper.berkeley.edu/wiki/Adder_tree'')')
      mask StyleString: edit,edit,popup(Behavioral|Fabric|DSP48),checkbox
  adder_tree2 : Subsystem  AncestorBlock=casper_library_misc/adder_tree  mask(adder_tree){n_inputs=4, latency=1, adder_imp=Fabric, first_stage_hdl=off}
      mask prompts: n_inputs "Number of Inputs"; latency "Add Latency"; adder_imp "Adder implementation"; first_stage_hdl "Use behavioural HDL for first stage of adders"
      mask help:
      | Sums all inputs using a tree of adds and delays.
      |
      | Number of inputs: The number of inputs to the block to be summed
      | Add latency: The number of clock cycles to perform one addition (affects timing)..
      | Adder implementation: choice of fabric or DSP48E core, or behavioral HDL
      | Use behavioural HDL for first stage of adders: Causes the first stage of adders to be absorbed into DSP blocks if multipliers precede them (Virtex 5). Overrides Adder implementation
      mask init:
      | adder_tree_init(gcb, ...
      |     'n_inputs', n_inputs, ...
      |     'latency', latency, ...
      |     'adder_imp', adder_imp, ...
      |     'first_stage_hdl', first_stage_hdl);
      settings: AttributesFormatString=latency 2
      mask Help: eval('xlWeb(''http://casper.berkeley.edu/wiki/Adder_tree'')')
      mask StyleString: edit,edit,popup(Behavioral|Fabric|DSP48),checkbox
  convert1 : xbsIndex_r4/Convert  gui_display_data_type=Fixed-point  arith_type="Signed  (2's comp)"  n_bits=18  bin_pt=17  float_type=Single  exp_bits=8  fraction_bits=24  quantization=Truncate  overflow=Saturate  en=off  latency=1  dbl_ovrd=off  pipeline=on  block_type=convert
      settings: block_version=11.4
  convert2 : xbsIndex_r4/Convert  gui_display_data_type=Fixed-point  arith_type="Signed  (2's comp)"  n_bits=18  bin_pt=17  float_type=Single  exp_bits=8  fraction_bits=24  quantization=Truncate  overflow=Saturate  en=off  latency=1  dbl_ovrd=off  pipeline=off  block_type=convert
      settings: block_version=11.4
  delay1 : xbsIndex_r4/Delay  rst=off  infoeditControl=Selection of Reset will increase slice count due to use of real FFs and instead of SRLs  en=off  latency=1  dbl_ovrd=off  reg_retiming=off  block_type=delay
      settings: block_version=11.4
  ri_to_c : casper_library_misc/ri_to_c
  scale1 : xbsIndex_r4/Scale  scale_factor=-3  dbl_ovrd=off  block_type=scale
  scale2 : xbsIndex_r4/Scale  scale_factor=-3  dbl_ovrd=off  block_type=scale
  dout : Outport
  sync_out : Outport  Port=2
  wires:
  adder_tree1/2(dout) -> scale1/1
  scale1/1 -> convert1/1
  adder_tree2/2(dout) -> scale2/1
  scale2/1 -> convert2/1
  convert1/1 -> ri_to_c/1
  convert2/1 -> ri_to_c/2
  ri_to_c/1 -> dout/1
  sync/1 -> adder_tree1/1(sync), adder_tree2/1(sync)
  adder_tree1/1(sync_out) -> delay1/1
  delay1/1 -> sync_out/1
  din/1 -> Slice0_1/1, Slice0_2/1, Slice1_1/1, Slice1_2/1, Slice2_1/1, Slice2_2/1, Slice3_1/1, Slice3_2/1
  Slice0_1/1 -> Reint0_1/1
  Reint0_1/1 -> adder_tree1/2(din1)
  Slice0_2/1 -> Reint0_2/1
  Reint0_2/1 -> adder_tree2/2(din1)
  Slice1_1/1 -> Reint1_1/1
  Reint1_1/1 -> adder_tree1/3(din2)
  Slice1_2/1 -> Reint1_2/1
  Reint1_2/1 -> adder_tree2/3(din2)
  Slice2_1/1 -> Reint2_1/1
  Reint2_1/1 -> adder_tree1/4(din3)
  Slice2_2/1 -> Reint2_2/1
  Reint2_2/1 -> adder_tree2/4(din3)
  Slice3_1/1 -> Reint3_1/1
  Reint3_1/1 -> adder_tree1/5(din4)
  Slice3_2/1 -> Reint3_2/1
  Reint3_2/1 -> adder_tree2/5(din4)

== system casper_library_pfbs/last_tap/ri_to_c ==
  re : Inport
  im : Inport  Port=2
  Concat : xbsIndex_r4/Concat  num_inputs=2  dbl_ovrd=off  block_type=concat
      settings: block_version=9.1.01
  Reinterpret : xbsIndex_r4/Reinterpret  force_arith_type=on  arith_type=Unsigned  force_bin_pt=on  bin_pt=0  block_type=reinterpret
      settings: infoedit="Changes signal type without altering the binary representation.   You can changed the signal between signed and unsigned, and relocate the binary point.<P><P>Hardware notes: In hardware this block costs nothing.<P><P>Example:  Suppose the input is 6 bits wide, signed, with 2 fractional bits, and the output is forced to unsigned with 0 fractional bits.  Then an input of -2.0 (1110.00 in binary 2's complement) becomes an output of 56 (111000 in binary)."  block_version=9.1.01
  Reinterpret1 : xbsIndex_r4/Reinterpret  force_arith_type=on  arith_type=Unsigned  force_bin_pt=on  bin_pt=0  block_type=reinterpret
      settings: infoedit="Changes signal type without altering the binary representation.   You can changed the signal between signed and unsigned, and relocate the binary point.<P><P>Hardware notes: In hardware this block costs nothing.<P><P>Example:  Suppose the input is 6 bits wide, signed, with 2 fractional bits, and the output is forced to unsigned with 0 fractional bits.  Then an input of -2.0 (1110.00 in binary 2's complement) becomes an output of 56 (111000 in binary)."  block_version=9.1.01
  c : Outport
  wires:
  Reinterpret/1 -> Concat/1
  Reinterpret1/1 -> Concat/2
  re/1 -> Reinterpret/1
  Concat/1 -> c/1
  im/1 -> Reinterpret1/1
